simulink model "que_02"  (R2025a)
settings: Solver=VariableStepAuto  StartTime=0.0  StopTime=10.0  RelTol=1e-3
settings Model: Creator=nikul  LastModifiedBy=nikul

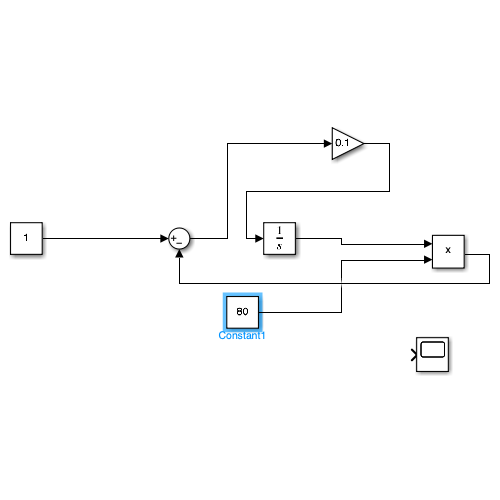
[thumbnail: Simulink's stored preview of the top-level diagram]
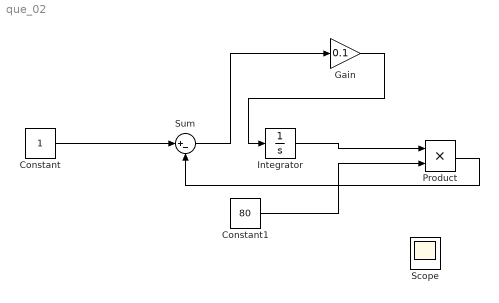
== system que_02 ==
  Constant : Constant
  Constant1 : Constant  Value=80
  Gain : Gain  Gain=0.1
  Integrator : Integrator
  Product : Product
  Scope : Scope
  Sum : Sum  Inputs=|+-
  wires:
  Constant/1 -> Sum/1
  Constant1/1 -> Product/2
  Integrator/1 -> Product/1
  Product/1 -> Sum/2
  Sum/1 -> Gain/1
  Gain/1 -> Integrator/1
